simulink model "Assignment_2_Spatial_Robotics"  (R2024b)
settings: Solver=ode4  StartTime=0.0  StopTime=inf  FixedStep=0.01  RelTol=1e-3  EnableMultiTasking=on
libraries: sharedutil x10, vrlib x3, matrix_library x1
settings Model: Creator=Member  LastModifiedBy=adyak
settings SolverCC: AlgebraicLoopSolver=TrustRegion
settings DataIOCC: LimitDataPoints=on  SaveFormat=Array  SignalLoggingSaveFormat=ModelDataLogs  SaveOutput=off  SignalLogging=off  SaveTime=off  ReturnWorkspaceOutputs=off
settings OptimizationCC: ExpressionDepthLimit=2147483647  InitFltsAndDblsToZero=on  LifeSpan=inf
settings DebuggingCC: ReadBeforeWriteMsg=DisableAll  WriteAfterWriteMsg=DisableAll  WriteAfterReadMsg=DisableAll  SaveWithParameterizedLinksMsg=none  UnderspecifiedInitializationDetection=Classic  MergeDetectMultiDrivingBlocksExec=none  SolverPrmCheckMsg=warning  MultiTaskDSMMsg=none  MultiTaskCondExecSysMsg=none  FcnCallInpInsideContextMsg=warning  UnconnectedInputMsg=warning  UnconnectedOutputMsg=warning  UnconnectedLineMsg=warning  StateNameClashWarn=warning  SFUnexpectedBacktrackingDiag=warning  SFNoUnconditionalDefaultTransitionDiag=warning  SFExecutionAtInitializationDiag=none  ArithmeticOperatorsInVariantConditions=warning
settings HardwareCC: ProdBitPerPointer=32  ProdBitPerSizeT=32  ProdBitPerPtrDiffT=32  ProdLargestAtomicFloat=None  ProdIntDivRoundTo=Undefined  ProdEndianess=Unspecified  ProdWordSize=32  ProdHWDeviceType=32-bit Generic
settings ModelReferenceCC: UpdateModelReferenceTargets=IfOutOfDate  EnableRefExpFcnMdlSchedulingChecks=on  PropagateSignalLabelsOutOfModel=off
settings SFSimCC: SFSimEcho=off  CustomCodeUndefinedFunction=UseInterfaceOnly
settings RTWCC: GPUComputeCapability=3.5
settings CodeAppCC: StateflowObjectComments=on
settings GRTTargetCC: TargetFcnLib=ansi_tfl_tmw.mat  TargetLangStandard=C89/C90 (ANSI)  CombineOutputUpdateFcns=off  GRTInterface=on
settings ConfigComp: CovMetricSettings=dw  CovSaveCumulativeToWorkspaceVar=on  CovSaveSingleToWorkspaceVar=on

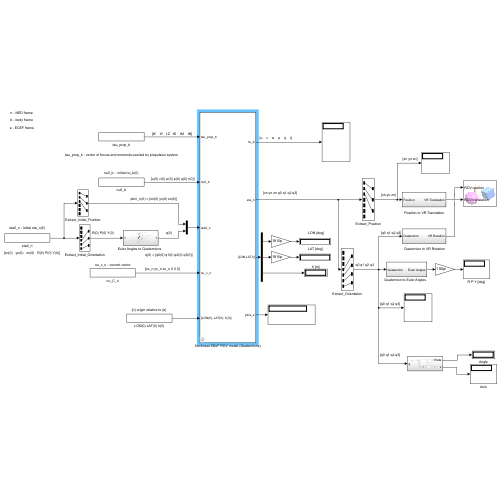
[thumbnail: Simulink's stored preview of the top-level diagram]
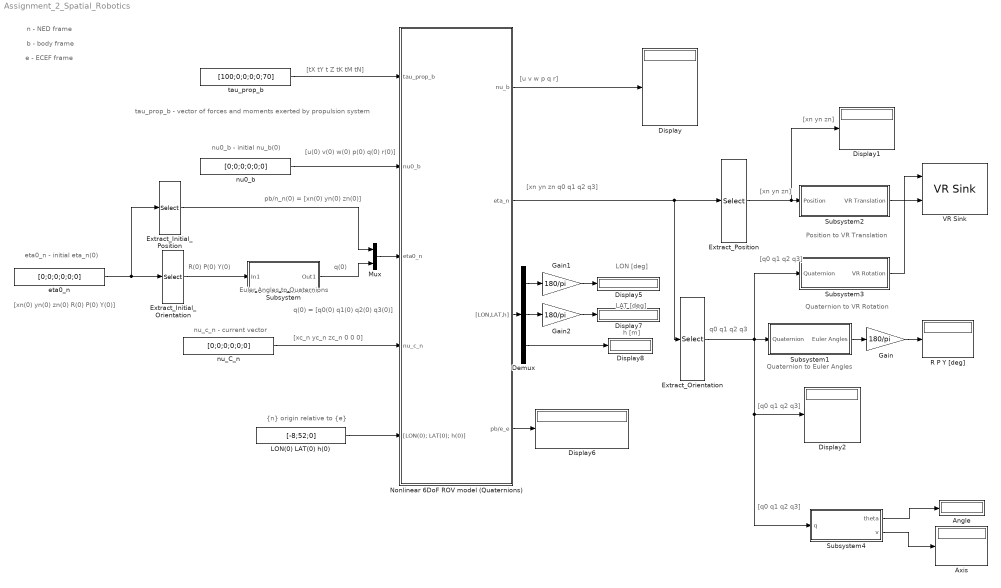
== system Assignment_2_Spatial_Robotics ==
  note: h [m]
  note: LON [deg]
  note: {n} origin relative to {e}
  note: q0 q1 q2 q3
  note: [xn yn zn]
  note: [xc_n yc_n zc_n 0 0 0]
  note: q(0)
  note: q(0) = [q0(0) q1(0) q2(0) q3(0)]
  note: pb/n_n(0) = [xn(0) yn(0) zn(0)]
  note: [u(0) v(0) w(0) p(0) q(0) r(0)]
  note: e - ECEF frame
  note: b - body frame
  note: n - NED frame
  note: tau_prop_b - vector of forces and moments exerted by propulsion system
  note: nu0_b - initial nu_b(0)
  note: eta0_n - initial eta_n(0)
  note: nu_c_n - current vector
  note: [tX tY t Z tK tM tN]
  note: [xn(0) yn(0) zn(0) R(0) P(0) Y(0)]
  note: [u v w p q r]
  note: [xn yn zn q0 q1 q2 q3]
  note: Euler Angles to Quaternions
  note: Quaternion to Euler Angles
  note: Quaternion to VR Rotation
  note: Position to VR Translation
  note: R(0) P(0) Y(0)
  note: [q0 q1 q2 q3]
  note: [xn yn zn]
  note: [q0 q1 q2 q3]
  note: [q0 q1 q2 q3]
  note: LAT [deg]
  Angle : Display
  Axis : Display
  Demux : Demux  Outputs=3
  Display{,1..2,5..8} (7 alike) : Display
  Extract_Initial_Orientation : Selector  InputPortWidth=6  IndexOptions=Index vector (dialog)  Indices=[4 5 6]  OutputSizes=1
  Extract_Initial_Position : Selector  InputPortWidth=6  IndexOptions=Index vector (dialog)  Indices=[1 2 3]  OutputSizes=1
  Extract_Orientation : Selector  InputPortWidth=7  IndexOptions=Index vector (dialog)  Indices=[4 5 6 7]  OutputSizes=1
  Extract_Position : Selector  InputPortWidth=7  IndexOptions=Index vector (dialog)  Indices=[1 2 3]  OutputSizes=1
  Gain : Gain  Gain=180/pi
  Gain1 : Gain  Gain=180/pi
  Gain2 : Gain  Gain=180/pi
  LON(0) LAT(0) h(0) : Constant  Value=[-8;52;0]
  Mux : Mux  Inputs=2
  Nonlinear 6DoF ROV model (Quaternions) : Subsystem  mask{Ig=[25 10 10;10 50 10;10 10 50], m=50, W=500, B=500, rG_b=[0;0;0], rB_b=[0;0;-0.1], MA=-diag([-30;-80;-80;-15;-30;-30]), DL=-diag([-200;-200;-200;-400;-300;-300]), dQ=-([-20;-20;-20;-10;-10;-10])}
      mask prompts: Ig "Inertia Tensor:"; m "Mass:"; W "Weigth:"; B "Buoyancy:"; MA "Added Mass Matrix MA:"; DL "Linear Damping Matrix DL:"; dQ "Quadratic Damping Vector dQ:"
      mask init:
      | Ib = Ig-m*skewsymm(rG_b)*skewsymm(rG_b);
      | MRB = [m*eye(3,3) -m*skewsymm(rG_b); m*skewsymm(rG_b) Ib];
      | M = MRB + MA;
      | inv_M = inv(M);
      | M11=MA(1:3,1:3);    M12=MA(1:3,4:6);
      | M21=MA(4:6,1:3);    M22=MA(4:6,4:6);
  R P Y [deg] : Display
  Subsystem : Subsystem
  Subsystem1 : Subsystem
  Subsystem2 : Subsystem
  Subsystem3 : Subsystem
  Subsystem4 : Subsystem
  VR Sink : vrlib/VR Sink  InstantiateOnLoad=on  SampleTime=-1  ViewEnable=on  RemoteChange=off  RemoteView=on  FieldsWritten=ROV.rotation.4.1.1.double#ROV.translation.3.1.1.double  WorldFileName=FALCON_test.wrl  AutoView=off  VideoDimensions=[]  AllowVariableSize=off  FigureProperties="{'Position', 'Name', 'Viewpoint', 'CameraBound', 'CameraDirection', 'CameraPosition', 'CameraUpVector', 'ZoomFactor', 'Antialiasing', 'Headlight', 'Lighting', 'Sound', 'StatusBar', 'Stereo3D', 'Stereo3DCameraOffset', 'Stereo3DHIT', 'ToolBar', 'Textures', 'Transparency', 'Triad', 'Wireframe', 'NavZones', 'NavMode', 'NavSpeed', 'CaptureFileFormat', 'CaptureFileName', 'Record2DCompressMethod', 'Record2DCompressQuality', 'Record2D', 'Record2DFileName', 'Record2DFPS', 'NavPanel'; [5.5850000000000000e+03   1.9000000000000000e+02   5.7600000000000000e+02   3.5000000000000000e+02], '', 'ONBOARD_CAMERA', 'on', [0.0000000000000000e+00   0.0000000000000000e+00  -1.0000000000000000e+00], [0.0000000000000000e+00   0.0000000000000000e+00   0.0000000000000000e+00], [0.0000000000000000e+00   1.0000000000000000e+00   0.0000000000000000e+00], [1.0000000000000000e+00], 'on', 'on', 'on', 'on', 'on', 'off', [1.0000000149011612e-01], [0.0000000000000000e+00], 'on', 'on', 'on', 'none', 'off', 'off', 'fly', 'normal', 'tif', '%f_anim_%n.tif', 'auto', [7.5000000000000000e+01], 'off', '%f_anim_%n.avi', 'auto', 'halfbar'}"
  eta0_n : Constant  Value=[0;0;0;0;0;0]
  nu0_b : Constant  Value=[0;0;0;0;0;0]
  nu_C_n : Constant  Value=[0;0;0;0;0;0]
  tau_prop_b : Constant  Value=[100;0;0;0;0;70]
  wires:
  nu0_b/1 -> Nonlinear 6DoF ROV model (Quaternions)/2(nu0_b)
  nu_C_n/1 -> Nonlinear 6DoF ROV model (Quaternions)/4(nu_c_n)
  tau_prop_b/1 -> Nonlinear 6DoF ROV model (Quaternions)/1(tau_prop_b)
  Nonlinear 6DoF ROV model (Quaternions)/2(eta_n) -> Extract_Orientation/1, Extract_Position/1
  Extract_Orientation/1 -> Subsystem4/1(q), Display2/1, Subsystem3/1(Quaternion), Subsystem1/1(Quaternion)
  Subsystem1/1(Euler Angles) -> Gain/1
  Gain/1 -> R P Y [deg]/1
  eta0_n/1 -> Extract_Initial_Position/1, Extract_Initial_Orientation/1
  Extract_Initial_Orientation/1 -> Subsystem/1(In1)
  Mux/1 -> Nonlinear 6DoF ROV model (Quaternions)/3(eta0_n)
  Subsystem/1(Out1) -> Mux/2
  Extract_Initial_Position/1 -> Mux/1
  Extract_Position/1 -> Display1/1, Subsystem2/1(Position)
  Subsystem3/1(VR Rotation) -> VR Sink/1
  Subsystem2/1(VR Translation) -> VR Sink/2
  Nonlinear 6DoF ROV model (Quaternions)/1(nu_b) -> Display/1
  Nonlinear 6DoF ROV model (Quaternions)/4(pb/e_e) -> Display6/1
  LON(0) LAT(0) h(0)/1 -> Nonlinear 6DoF ROV model (Quaternions)/5("[LON(0); LAT(0); h(0)]")
  Nonlinear 6DoF ROV model (Quaternions)/3("[LON,LAT,h]") -> Demux/1
  Demux/1 -> Gain1/1
  Gain1/1 -> Display5/1
  Gain2/1 -> Display7/1
  Demux/2 -> Gain2/1
  Demux/3 -> Display8/1
  Subsystem4/1(theta) -> Angle/1
  Subsystem4/2(v) -> Axis/1

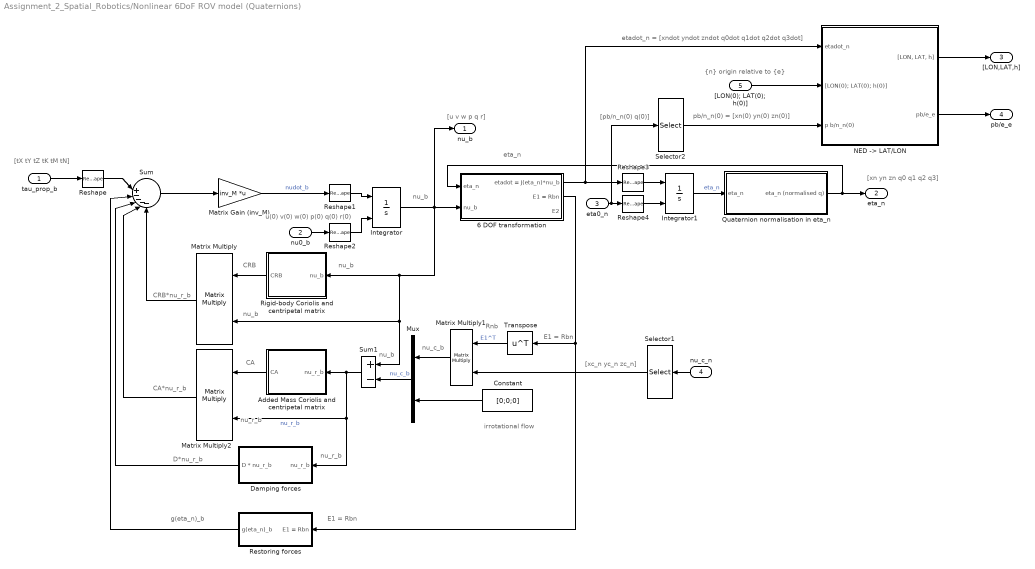
== system Assignment_2_Spatial_Robotics/Nonlinear 6DoF ROV model (Quaternions) ==
  note: irrotational flow
  note: etadot_n = [xndot yndot zndot q0dot q1dot q2dot q3dot]
  note: CA*nu_r_b
  note: D*nu_r_b
  note: g(eta_n)_b
  note: CRB
  note: CA
  note: u(0) v(0) w(0) p(0) q(0) r(0)
  note: eta_n
  note: [xn yn zn q0 q1 q2 q3]
  note: nu_r_b
  note: nu_c_b
  note: [xc_n yc_n zc_n]
  note: Rnb
  note: [tX tY tZ tK tM tN]
  note: [u v w p q r]
  note: nu_b
  note: E1 = Rbn
  note: nu_b
  note: nu_b
  note: nu_b
  note: nu_r_b
  note: CRB*nu_r_b
  note: pb/n_n(0) = [xn(0) yn(0) zn(0)]
  note: [pb/n_n(0) q(0)]
  note: {n} origin relative to {e}
  note: E1 = Rbn
  tau_prop_b : Inport
  nu0_b : Inport  Port=2
  eta0_n : Inport  Port=3
  nu_c_n : Inport  Port=4
  "[LON(0); LAT(0); h(0)]" : Inport  Port=5
  6 DOF transformation : Subsystem  AncestorBlock=MarineGNC/Library blocks/Axes transformations/6 DOF transformation
  Added Mass Coriolis and centripetal matrix : Subsystem
  Constant : Constant  Value=[0;0;0]
  Damping forces : Subsystem
  Integrator : Integrator  InitialConditionSource=external
  Integrator1 : Integrator  InitialConditionSource=external
  Matrix Gain (inv_M) : Gain  Gain=inv_M  Multiplication=Matrix(K*u)  SaturateOnIntegerOverflow=on  OutDataTypeStr=Inherit: Same as input  ParamDataTypeStr=Inherit: Same as input
  Matrix Multiply : Product  Multiplication=Matrix(*)
  Matrix Multiply1 : Product  Multiplication=Matrix(*)
  Matrix Multiply2 : Product  Multiplication=Matrix(*)
  Mux : Mux  Inputs=2
  "NED -> LAT/LON" : Subsystem
  Quaternion normalisation in eta_n : Subsystem
  Reshape{,1..4} (5 alike) : Reshape  OutputDimensionality=Column vector (2-D)
  Restoring forces : Subsystem
  Rigid-body Coriolis and centripetal matrix : Subsystem
  Selector1 : Selector  InputPortWidth=6  IndexOptions=Index vector (dialog)  Indices=[1 2 3]  OutputSizes=1
  Selector2 : Selector  InputPortWidth=7  IndexOptions=Index vector (dialog)  Indices=[1 2 3]  OutputSizes=1
  Sum : Sum  Inputs=|||+----  SaturateOnIntegerOverflow=on
  Sum1 : Sum  Inputs=+-
  Transpose : Math  Operator=transpose  SignedPower=on
  nu_b : Outport  VectorParamsAs1DForOutWhenUnconnected=off
  eta_n : Outport  Port=2  VectorParamsAs1DForOutWhenUnconnected=off
  "[LON,LAT,h]" : Outport  Port=3  VectorParamsAs1DForOutWhenUnconnected=off
  pb/e_e : Outport  Port=4  VectorParamsAs1DForOutWhenUnconnected=off
  wires:
  Matrix Multiply2/1 -> Sum/4
  Added Mass Coriolis and centripetal matrix/1(CA) -> Matrix Multiply2/1
  Sum1/1 -> Damping forces/1(nu_r_b), Matrix Multiply2/2, Added Mass Coriolis and centripetal matrix/1(nu_r_b)  "nu_r_b"
  Transpose/1 -> Matrix Multiply1/1  "E1^T"
  Matrix Multiply/1 -> Sum/5
  Rigid-body Coriolis and centripetal matrix/1(CRB) -> Matrix Multiply/1
  Reshape4/1 -> Integrator1/2
  Reshape3/1 -> Integrator1/1
  Reshape2/1 -> Integrator/2
  Reshape1/1 -> Integrator/1
  Reshape/1 -> Sum/1
  Restoring forces/1(g(eta_n)_b) -> Sum/2
  Damping forces/1(D * nu_r_b) -> Sum/3
  eta0_n/1 -> Selector2/1, Reshape4/1
  6 DOF transformation/1(etadot = J(eta_n)*nu_b) -> "NED -> LAT/LON"/1(etadot_n), Reshape3/1
  Integrator/1 -> 6 DOF transformation/2(nu_b), nu_b/1, Rigid-body Coriolis and centripetal matrix/1(nu_b), Matrix Multiply/2, Sum1/1
  nu0_b/1 -> Reshape2/1
  Matrix Gain (inv_M)/1 -> Reshape1/1  "nudot_b"
  Sum/1 -> Matrix Gain (inv_M)/1
  tau_prop_b/1 -> Reshape/1
  Matrix Multiply1/1 -> Mux/1
  Mux/1 -> Sum1/2  "nu_c_b"
  nu_c_n/1 -> Selector1/1
  Selector1/1 -> Matrix Multiply1/2
  6 DOF transformation/2(E1 = Rbn) -> Transpose/1, Restoring forces/1(E1 = Rbn)
  Integrator1/1 -> Quaternion normalisation in eta_n/1(eta_n)  "eta_n"
  Quaternion normalisation in eta_n/1(eta_n (normalised q)) -> 6 DOF transformation/1(eta_n), eta_n/1
  Constant/1 -> Mux/2
  Selector2/1 -> "NED -> LAT/LON"/3(p b/n_n(0))
  "[LON(0); LAT(0); h(0)]"/1 -> "NED -> LAT/LON"/2("[LON(0); LAT(0); h(0)]")
  "NED -> LAT/LON"/1("[LON, LAT, h]") -> "[LON,LAT,h]"/1
  "NED -> LAT/LON"/2(pb/e_e) -> pb/e_e/1

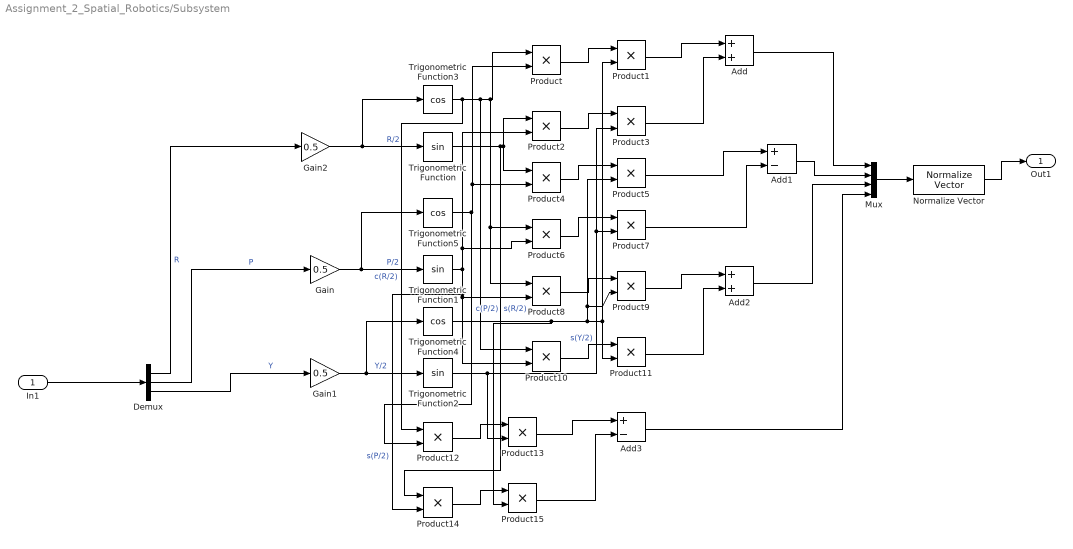
== system Assignment_2_Spatial_Robotics/Subsystem ==
  In1 : Inport
  Add : Sum
  Add1 : Sum  Inputs=+-
  Add2 : Sum
  Add3 : Sum  Inputs=+-
  Demux : Demux  Outputs=3
  Gain : Gain  Gain=0.5
  Gain1 : Gain  Gain=0.5
  Gain2 : Gain  Gain=0.5
  Mux : Mux
  Normalize Vector : vrlib/Utilities/Normalize Vector  maxzero=0
  Product{,1..15} (16 alike) : Product
  Trigonometric Function : Trigonometry
  Trigonometric Function1 : Trigonometry
  Trigonometric Function2 : Trigonometry
  Trigonometric Function3 : Trigonometry  Operator=cos
  Trigonometric Function4 : Trigonometry  Operator=cos
  Trigonometric Function5 : Trigonometry  Operator=cos
  Out1 : Outport
  wires:
  In1/1 -> Demux/1
  Demux/3 -> Gain1/1  "Y"
  Demux/2 -> Gain/1  "P"
  Demux/1 -> Gain2/1  "R"
  Gain1/1 -> Trigonometric Function4/1, Trigonometric Function2/1  "Y/2"
  Gain/1 -> Trigonometric Function5/1, Trigonometric Function1/1  "P/2"
  Gain2/1 -> Trigonometric Function3/1, Trigonometric Function/1  "R/2"
  Trigonometric Function/1 -> Product14/1, Product2/1, Product4/1  "s(R/2)"
  Trigonometric Function1/1 -> Product14/2, Product10/2, Product8/2, Product6/2, Product2/2  "s(P/2)"
  Product/1 -> Product1/1
  Trigonometric Function2/1 -> Product13/2, Product7/2, Product3/2  "s(Y/2)"
  Trigonometric Function3/1 -> Product12/1, Product10/1, Product8/1, Product6/1, Product/1  "c(R/2)"
  Trigonometric Function5/1 -> Product12/2, Product4/2, Product/2  "c(P/2)"
  Trigonometric Function4/1 -> Product15/2, Product9/2, Product5/2, Product11/2, Product1/2
  Product1/1 -> Add/1
  Product3/1 -> Add/2
  Product2/1 -> Product3/1
  Product5/1 -> Add1/1
  Product4/1 -> Product5/1
  Product7/1 -> Add1/2
  Product6/1 -> Product7/1
  Product9/1 -> Add2/1
  Product8/1 -> Product9/1
  Product11/1 -> Add2/2
  Product10/1 -> Product11/1
  Product13/1 -> Add3/1
  Product12/1 -> Product13/1
  Product15/1 -> Add3/2
  Product14/1 -> Product15/1
  Add/1 -> Mux/1
  Add1/1 -> Mux/2
  Add2/1 -> Mux/3
  Add3/1 -> Mux/4
  Mux/1 -> Normalize Vector/1
  Normalize Vector/1 -> Out1/1

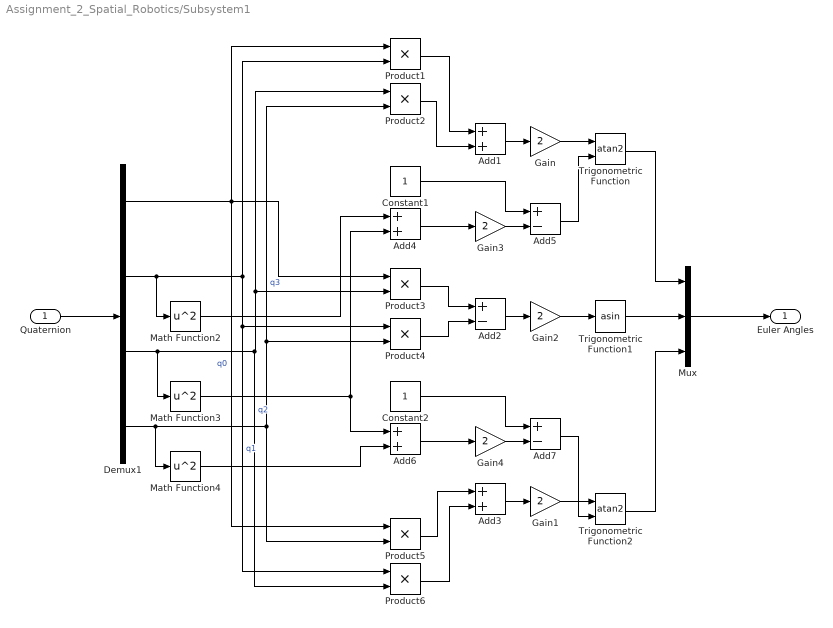
== system Assignment_2_Spatial_Robotics/Subsystem1 ==
  Quaternion : Inport
  Add{1,3..4,6} (4 alike) : Sum
  Add2 : Sum  Inputs=+-
  Add5 : Sum  Inputs=+-
  Add7 : Sum  Inputs=+-
  Constant1 : Constant
  Constant2 : Constant
  Demux1 : Demux
  Gain{,1..4} (5 alike) : Gain  Gain=2
  Math Function2 : Math  Operator=square  SignedPower=on
  Math Function3 : Math  Operator=square  SignedPower=on
  Math Function4 : Math  Operator=square  SignedPower=on
  Mux : Mux  Inputs=3
  Product{1..6} (6 alike) : Product
  Trigonometric Function : Trigonometry  Operator=atan2
  Trigonometric Function1 : Trigonometry  Operator=asin
  Trigonometric Function2 : Trigonometry  Operator=atan2
  Euler Angles : Outport  VectorParamsAs1DForOutWhenUnconnected=off
  wires:
  Quaternion/1 -> Demux1/1
  Demux1/1 -> Product5/1, Product3/1, Product1/1  "q0"
  Demux1/2 -> Product6/1, Product4/1, Product1/2, Math Function2/1  "q1"
  Demux1/3 -> Product6/2, Product3/2, Product2/1, Math Function3/1  "q2"
  Demux1/4 -> Product5/2, Product4/2, Product2/2, Math Function4/1  "q3"
  Trigonometric Function1/1 -> Mux/2
  Mux/1 -> Euler Angles/1
  Trigonometric Function/1 -> Mux/1
  Trigonometric Function2/1 -> Mux/3
  Gain/1 -> Trigonometric Function/1
  Gain1/1 -> Trigonometric Function2/1
  Gain2/1 -> Trigonometric Function1/1
  Add1/1 -> Gain/1
  Add2/1 -> Gain2/1
  Add3/1 -> Gain1/1
  Product3/1 -> Add2/1
  Product4/1 -> Add2/2
  Product5/1 -> Add3/1
  Product6/1 -> Add3/2
  Product2/1 -> Add1/2
  Product1/1 -> Add1/1
  Add4/1 -> Gain3/1
  Gain3/1 -> Add5/2
  Constant1/1 -> Add5/1
  Add5/1 -> Trigonometric Function/2
  Add7/1 -> Trigonometric Function2/2
  Add6/1 -> Gain4/1
  Gain4/1 -> Add7/2
  Constant2/1 -> Add7/1
  Math Function2/1 -> Add4/1
  Math Function3/1 -> Add6/1, Add4/2
  Math Function4/1 -> Add6/2

== system Assignment_2_Spatial_Robotics/Subsystem2 ==
  Position : Inport
  Demux : Demux  Outputs=3
  Gain : Gain  Gain=-1
  Gain1 : Gain  Gain=-1
  Mux : Mux  Inputs=3
  VR Translation : Outport  VectorParamsAs1DForOutWhenUnconnected=off
  wires:
  Position/1 -> Demux/1
  Demux/1 -> Gain/1  "x"
  Demux/2 -> Mux/1  "y"
  Demux/3 -> Gain1/1  "z"
  Mux/1 -> VR Translation/1
  Gain1/1 -> Mux/2
  Gain/1 -> Mux/3

== system Assignment_2_Spatial_Robotics/Subsystem3 ==
  Quaternion : Inport
  Demux1 : Demux
  Gain : Gain  Gain=2
  Gain1 : Gain  Gain=-1
  Gain2 : Gain  Gain=-1
  Mux : Mux
  Trigonometric Function : Trigonometry  Operator=acos
  VR Rotation : Outport  VectorParamsAs1DForOutWhenUnconnected=off
  wires:
  Trigonometric Function/1 -> Gain/1
  Gain/1 -> Mux/4
  Mux/1 -> VR Rotation/1
  Demux1/1 -> Trigonometric Function/1  "q0"
  Demux1/2 -> Gain1/1  "q1"
  Demux1/3 -> Mux/1  "q2"
  Demux1/4 -> Gain2/1  "q3"
  Gain2/1 -> Mux/2
  Gain1/1 -> Mux/3
  Quaternion/1 -> Demux1/1

== system Assignment_2_Spatial_Robotics/Subsystem4 ==
  q : Inport
  Demux : Demux
  Gain : Gain  Gain=2
  Mux : Mux  Inputs=3
  Normalize Vector : vrlib/Utilities/Normalize Vector  maxzero=0
  Product : Product
  Trigonometric Function : Trigonometry  Operator=cos
  theta : Outport
  v : Outport  Port=2
  wires:
  q/1 -> Demux/1
  Demux/1 -> Trigonometric Function/1  "q0"
  Trigonometric Function/1 -> Product/1
  Gain/1 -> Product/2
  Demux/2 -> Mux/1  "q1"
  Demux/3 -> Mux/2  "q2"
  Demux/4 -> Mux/3  "q3"
  Mux/1 -> Normalize Vector/1
  Normalize Vector/1 -> v/1
  Product/1 -> theta/1

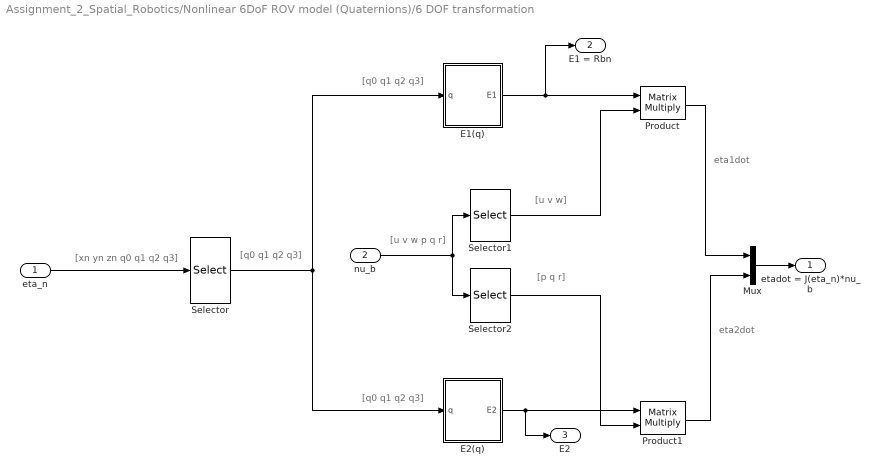
== system Assignment_2_Spatial_Robotics/Nonlinear 6DoF ROV model (Quaternions)/6 DOF transformation ==
  note: [u v w p q r]
  note: [q0 q1 q2 q3]
  note: [xn yn zn q0 q1 q2 q3]
  note: eta1dot
  note: eta2dot
  note: [q0 q1 q2 q3]
  note: [q0 q1 q2 q3]
  note: [u v w]
  note: [p q r]
  eta_n : Inport
  nu_b : Inport  Port=2
  E1(q) : Subsystem
  E2(q) : Subsystem
  Mux : Mux  Inputs=2
  Product : Product  Inputs=**  Multiplication=Matrix(*)  SaturateOnIntegerOverflow=on  OutDataTypeStr=Inherit: Same as first input
  Product1 : Product  Inputs=**  Multiplication=Matrix(*)  SaturateOnIntegerOverflow=on  OutDataTypeStr=Inherit: Same as first input
  Selector : Selector  InputPortWidth=7  IndexOptions=Index vector (dialog)  Indices=[4 5 6 7]  OutputSizes=1
  Selector1 : Selector  InputPortWidth=6  IndexOptions=Index vector (dialog)  Indices=[1 2 3]  OutputSizes=1
  Selector2 : Selector  InputPortWidth=6  IndexOptions=Index vector (dialog)  Indices=[4 5 6]  OutputSizes=1
  etadot = J(eta_n)*nu_b : Outport  VectorParamsAs1DForOutWhenUnconnected=off
  E1 = Rbn : Outport  Port=2  VectorParamsAs1DForOutWhenUnconnected=off
  E2 : Outport  Port=3  VectorParamsAs1DForOutWhenUnconnected=off
  wires:
  Product1/1 -> Mux/2
  Mux/1 -> etadot = J(eta_n)*nu_b/1
  Product/1 -> Mux/1
  E2(q)/1(E2) -> Product1/1, E2/1
  Selector2/1 -> Product1/2
  Selector1/1 -> Product/2
  nu_b/1 -> Selector2/1, Selector1/1
  E1(q)/1(E1) -> Product/1, E1 = Rbn/1
  eta_n/1 -> Selector/1
  Selector/1 -> E2(q)/1(q), E1(q)/1(q)

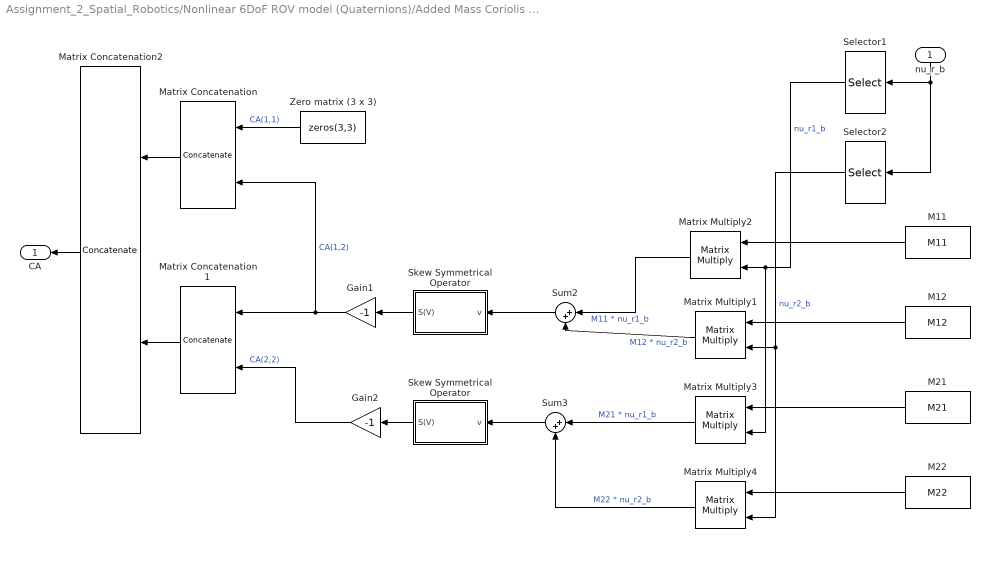
== system Assignment_2_Spatial_Robotics/Nonlinear 6DoF ROV model (Quaternions)/Added Mass Coriolis and centripetal matrix ==
  nu_r_b : Inport
  Gain1 : Gain  Gain=-1  SaturateOnIntegerOverflow=on  OutDataTypeStr=Inherit: Same as input  ParamDataTypeStr=Inherit: Same as input
  Gain2 : Gain  Gain=-1  SaturateOnIntegerOverflow=on  OutDataTypeStr=Inherit: Same as input  ParamDataTypeStr=Inherit: Same as input
  M11 : Constant  Value=M11
  M12 : Constant  Value=M12
  M21 : Constant  Value=M21
  M22 : Constant  Value=M22
  Matrix Concatenation : Concatenate  Mode=Multidimensional array
  Matrix Concatenation1 : Concatenate  Mode=Multidimensional array
  Matrix Concatenation2 : Concatenate  Mode=Multidimensional array  ConcatenateDimension=2
  Matrix Multiply{1..4} (4 alike) : Product  Multiplication=Matrix(*)
  Selector1 : Selector  InputPortWidth=6  IndexOptions=Index vector (dialog)  Indices=[1 2 3]  OutputSizes=1
  Selector2 : Selector  InputPortWidth=6  IndexOptions=Index vector (dialog)  Indices=[4 5 6]  OutputSizes=1
  Skew Symmetrical Operator : Subsystem
  "Skew Symmetrical Operator " : Subsystem
  Sum2 : Sum  Inputs=|++  SaturateOnIntegerOverflow=on
  Sum3 : Sum  Inputs=|++  SaturateOnIntegerOverflow=on
  Zero matrix (3 x 3) : Constant  Value=zeros(3,3)
  CA : Outport  VectorParamsAs1DForOutWhenUnconnected=off
  wires:
  Zero matrix (3 x 3)/1 -> Matrix Concatenation/1  "CA(1,1)"
  Matrix Concatenation/1 -> Matrix Concatenation2/1
  Matrix Concatenation1/1 -> Matrix Concatenation2/2
  Matrix Multiply2/1 -> Sum2/1  "M11 * nu_r1_b"
  Matrix Multiply1/1 -> Sum2/2  "M12 * nu_r2_b"
  Matrix Multiply3/1 -> Sum3/1  "M21 * nu_r1_b"
  Selector1/1 -> Matrix Multiply2/2, Matrix Multiply3/2  "nu_r1_b"
  Matrix Multiply4/1 -> Sum3/2  "M22 * nu_r2_b"
  Selector2/1 -> Matrix Multiply1/2, Matrix Multiply4/2  "nu_r2_b"
  Sum2/1 -> "Skew Symmetrical Operator "/1(v)
  Sum3/1 -> Skew Symmetrical Operator/1(v)
  "Skew Symmetrical Operator "/1(S(V)) -> Gain1/1
  Skew Symmetrical Operator/1(S(V)) -> Gain2/1
  Gain1/1 -> Matrix Concatenation1/1, Matrix Concatenation/2  "CA(1,2)"
  Gain2/1 -> Matrix Concatenation1/2  "CA(2,2)"
  nu_r_b/1 -> Selector1/1, Selector2/1
  Matrix Concatenation2/1 -> CA/1
  M11/1 -> Matrix Multiply2/1
  M12/1 -> Matrix Multiply1/1
  M21/1 -> Matrix Multiply3/1
  M22/1 -> Matrix Multiply4/1

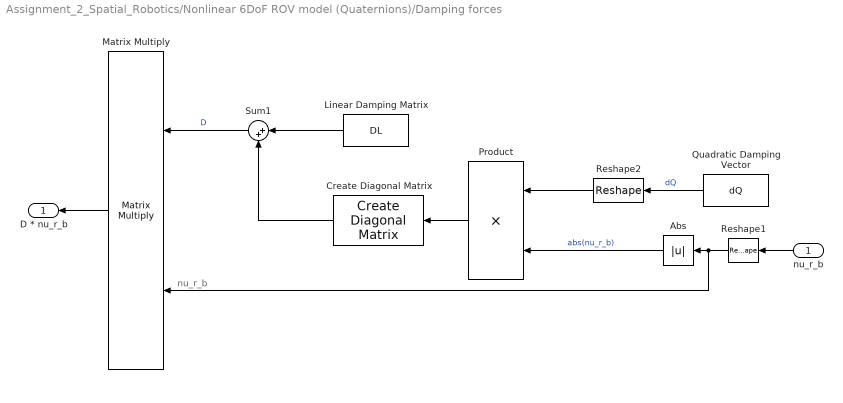
== system Assignment_2_Spatial_Robotics/Nonlinear 6DoF ROV model (Quaternions)/Damping forces ==
  note: nu_r_b
  nu_r_b : Inport
  Abs : Abs
  Create Diagonal Matrix : matrix_library/Create Diagonal Matrix
  Linear Damping Matrix : Constant  Value=DL
  Matrix Multiply : Product  Multiplication=Matrix(*)
  Product : Product  SaturateOnIntegerOverflow=on  OutDataTypeStr=Inherit: Same as first input
  Quadratic Damping Vector : Constant  Value=dQ
  Reshape1 : Reshape  OutputDimensionality=Column vector (2-D)
  Reshape2 : Reshape  OutputDimensionality=Column vector (2-D)  OutputDimensions=[6,6]
  Sum1 : Sum  Inputs=|++  SaturateOnIntegerOverflow=on
  D * nu_r_b : Outport  VectorParamsAs1DForOutWhenUnconnected=off
  wires:
  Reshape2/1 -> Product/1
  Reshape1/1 -> Matrix Multiply/2, Abs/1
  Matrix Multiply/1 -> D * nu_r_b/1
  Sum1/1 -> Matrix Multiply/1  "D"
  nu_r_b/1 -> Reshape1/1
  Linear Damping Matrix/1 -> Sum1/1
  Create Diagonal Matrix/1 -> Sum1/2
  Product/1 -> Create Diagonal Matrix/1
  Abs/1 -> Product/2  "abs(nu_r_b)"
  Quadratic Damping Vector/1 -> Reshape2/1  "dQ"

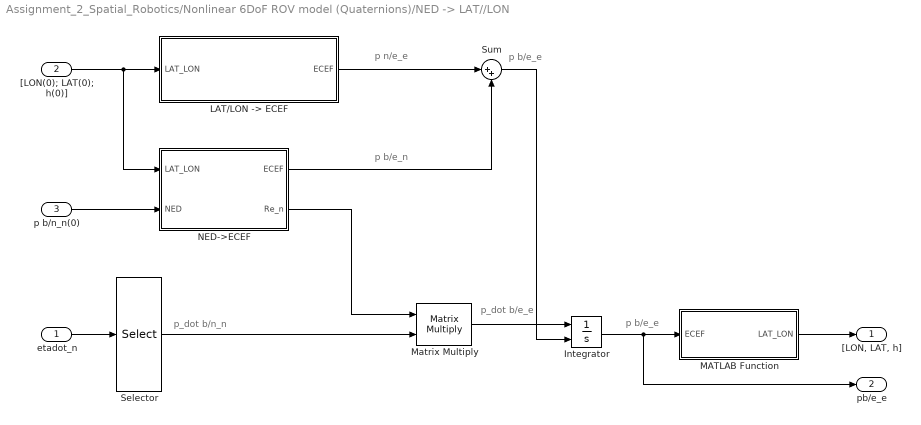
== system Assignment_2_Spatial_Robotics/Nonlinear 6DoF ROV model (Quaternions)/NED -> LAT//LON ==
  note: p_dot b/n_n
  note: p_dot b/e_e
  note: p b/e_e
  note: p n/e_e
  note: p b/e_n
  note: p b/e_e
  etadot_n : Inport
  "[LON(0); LAT(0); h(0)]" : Inport  Port=2
  p b/n_n(0) : Inport  Port=3
  Integrator : Integrator  InitialConditionSource=external
  "LAT/LON -> ECEF" : MATLAB Function  TreatAsAtomicUnit=on
  MATLAB Function : MATLAB Function  TreatAsAtomicUnit=on
  Matrix Multiply : Product  Multiplication=Matrix(*)
  NED->ECEF : MATLAB Function  TreatAsAtomicUnit=on
  Selector : Selector  InputPortWidth=7  IndexOptions=Index vector (dialog)  Indices=[1 2 3]  OutputSizes=1
  Sum : Sum  Inputs=|++
  "[LON, LAT, h]" : Outport
  pb/e_e : Outport  Port=2
  wires:
  etadot_n/1 -> Selector/1
  Selector/1 -> Matrix Multiply/2
  "[LON(0); LAT(0); h(0)]"/1 -> NED->ECEF/1(LAT_LON), "LAT/LON -> ECEF"/1(LAT_LON)
  Sum/1 -> Integrator/2
  Integrator/1 -> MATLAB Function/1(ECEF), pb/e_e/1
  MATLAB Function/1(LAT_LON) -> "[LON, LAT, h]"/1
  p b/n_n(0)/1 -> NED->ECEF/2(NED)
  Matrix Multiply/1 -> Integrator/1
  NED->ECEF/2(Re_n) -> Matrix Multiply/1
  NED->ECEF/1(ECEF) -> Sum/2
  "LAT/LON -> ECEF"/1(ECEF) -> Sum/1

== system Assignment_2_Spatial_Robotics/Nonlinear 6DoF ROV model (Quaternions)/Quaternion normalisation in eta_n ==
  note: q (normalised)
  note: q
  note: norm(q)
  note: q=[q0 q1 q2 q3]
  note: [xn yn zn]
  note: [xn yn zn q0 q1 q2 q3]
  eta_n : Inport
  Mux : Mux  Inputs=2
  Product : Product  Inputs=*/  SaturateOnIntegerOverflow=on  OutDataTypeStr=Inherit: Same as first input
  Reshape : Reshape  OutputDimensionality=Column vector (2-D)
  Selector : Selector  InputPortWidth=7  IndexOptions=Index vector (dialog)  Indices=[1 2 3]  OutputSizes=1
  Selector1 : Selector  InputPortWidth=7  IndexOptions=Index vector (dialog)  Indices=[4 5 6 7]  OutputSizes=1
  norm : MATLABFcn  MATLABFcn=norm  OutputDimensions=1
  eta_n (normalised q) : Outport  VectorParamsAs1DForOutWhenUnconnected=off
  wires:
  eta_n/1 -> Selector1/1, Selector/1
  Selector1/1 -> norm/1, Product/1
  norm/1 -> Product/2
  Selector/1 -> Mux/1
  Product/1 -> Mux/2
  Mux/1 -> Reshape/1
  Reshape/1 -> eta_n (normalised q)/1

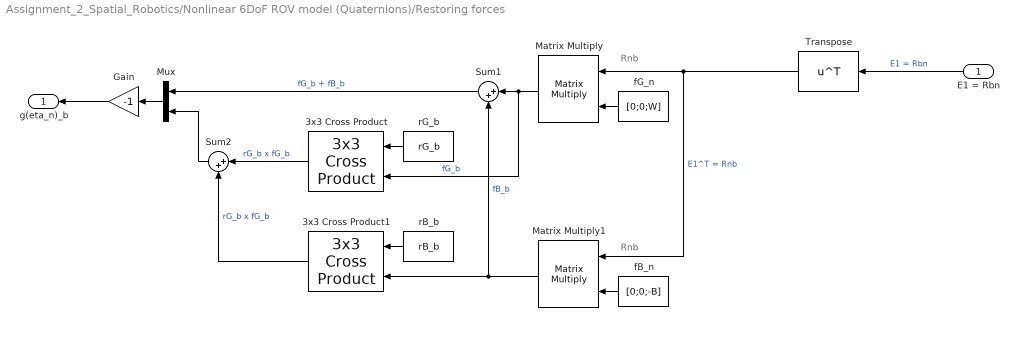
== system Assignment_2_Spatial_Robotics/Nonlinear 6DoF ROV model (Quaternions)/Restoring forces ==
  note: Rnb
  note: Rnb
  E1 = Rbn : Inport
  3x3 Cross Product : sharedutil/3x3 Cross Product  aMode=aMode
  3x3 Cross Product1 : sharedutil/3x3 Cross Product  aMode=aMode
  Gain : Gain  Gain=-1  SaturateOnIntegerOverflow=on  OutDataTypeStr=Inherit: Same as input  ParamDataTypeStr=Inherit: Same as input
  Matrix Multiply : Product  Multiplication=Matrix(*)
  Matrix Multiply1 : Product  Multiplication=Matrix(*)
  Mux : Mux  Inputs=2
  Sum1 : Sum  Inputs=|++  SaturateOnIntegerOverflow=on
  Sum2 : Sum  Inputs=|++  SaturateOnIntegerOverflow=on
  Transpose : Math  Operator=transpose  SignedPower=on
  fB_n : Constant  Value=[0;0;-B]
  fG_n : Constant  Value=[0;0;W]
  rB_b : Constant  Value=rB_b
  rG_b : Constant  Value=rG_b
  g(eta_n)_b : Outport  VectorParamsAs1DForOutWhenUnconnected=off
  wires:
  E1 = Rbn/1 -> Transpose/1  "E1 = Rbn"
  Transpose/1 -> Matrix Multiply/1, Matrix Multiply1/1  "E1^T = Rnb"
  fG_n/1 -> Matrix Multiply/2
  fB_n/1 -> Matrix Multiply1/2
  Matrix Multiply/1 -> Sum1/1, 3x3 Cross Product/2  "fG_b"
  Matrix Multiply1/1 -> Sum1/2, 3x3 Cross Product1/2  "fB_b"
  rG_b/1 -> 3x3 Cross Product/1
  Sum1/1 -> Mux/1  "fG_b + fB_b"
  3x3 Cross Product/1 -> Sum2/1  "rG_b x fG_b"
  3x3 Cross Product1/1 -> Sum2/2  "rG_b x fG_b"
  rB_b/1 -> 3x3 Cross Product1/1
  Sum2/1 -> Mux/2
  Mux/1 -> Gain/1
  Gain/1 -> g(eta_n)_b/1

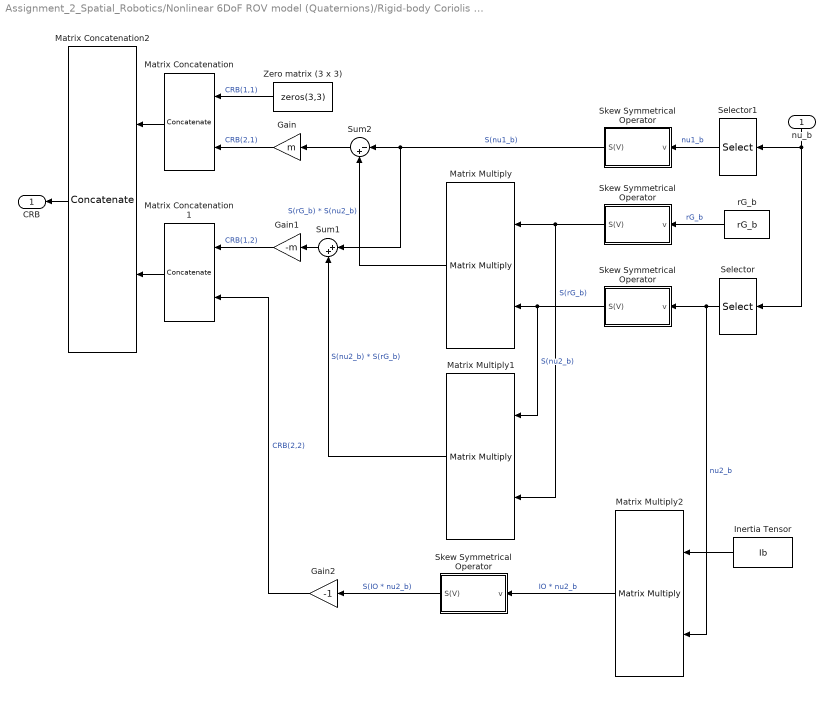
== system Assignment_2_Spatial_Robotics/Nonlinear 6DoF ROV model (Quaternions)/Rigid-body Coriolis and centripetal matrix ==
  nu_b : Inport
  Gain : Gain  Gain=m  SaturateOnIntegerOverflow=on  OutDataTypeStr=Inherit: Same as input  ParamDataTypeStr=Inherit: Same as input
  Gain1 : Gain  Gain=-m  SaturateOnIntegerOverflow=on  OutDataTypeStr=Inherit: Same as input  ParamDataTypeStr=Inherit: Same as input
  Gain2 : Gain  Gain=-1  SaturateOnIntegerOverflow=on  OutDataTypeStr=Inherit: Same as input  ParamDataTypeStr=Inherit: Same as input
  Inertia Tensor : Constant  Value=Ib
  Matrix Concatenation : Concatenate  Mode=Multidimensional array
  Matrix Concatenation1 : Concatenate  Mode=Multidimensional array
  Matrix Concatenation2 : Concatenate  Mode=Multidimensional array  ConcatenateDimension=2
  Matrix Multiply : Product  Multiplication=Matrix(*)
  Matrix Multiply1 : Product  Multiplication=Matrix(*)
  Matrix Multiply2 : Product  Multiplication=Matrix(*)
  Selector : Selector  InputPortWidth=6  IndexOptions=Index vector (dialog)  Indices=[4 5 6]  OutputSizes=1
  Selector1 : Selector  InputPortWidth=6  IndexOptions=Index vector (dialog)  Indices=[1 2 3]  OutputSizes=1
  "Skew Symmetrical Operator " : Subsystem
  Skew Symmetrical Operator : Subsystem
  "Skew Symmetrical Operator " : Subsystem
  "Skew Symmetrical Operator  " : Subsystem
  Sum1 : Sum  Inputs=|++  SaturateOnIntegerOverflow=on
  Sum2 : Sum  Inputs=|-+  SaturateOnIntegerOverflow=on
  Zero matrix (3 x 3) : Constant  Value=zeros(3,3)
  rG_b : Constant  Value=rG_b
  CRB : Outport  VectorParamsAs1DForOutWhenUnconnected=off
  wires:
  nu_b/1 -> Selector/1, Selector1/1
  Selector1/1 -> Skew Symmetrical Operator/1(v)  "nu1_b"
  Selector/1 -> "Skew Symmetrical Operator "/1(v), Matrix Multiply2/2  "nu2_b"
  rG_b/1 -> "Skew Symmetrical Operator  "/1(v)  "rG_b"
  Skew Symmetrical Operator/1(S(V)) -> Sum2/1, Sum1/1  "S(nu1_b)"
  "Skew Symmetrical Operator "/1(S(V)) -> Matrix Multiply/2, Matrix Multiply1/1  "S(nu2_b)"
  "Skew Symmetrical Operator  "/1(S(V)) -> Matrix Multiply/1, Matrix Multiply1/2  "S(rG_b)"
  Matrix Multiply/1 -> Sum2/2  "S(rG_b) * S(nu2_b)"
  Sum2/1 -> Gain/1
  Gain/1 -> Matrix Concatenation/2  "CRB(2,1)"
  Zero matrix (3 x 3)/1 -> Matrix Concatenation/1  "CRB(1,1)"
  Matrix Multiply1/1 -> Sum1/2  "S(nu2_b) * S(rG_b)"
  Sum1/1 -> Gain1/1
  Gain1/1 -> Matrix Concatenation1/1  "CRB(1,2)"
  Inertia Tensor/1 -> Matrix Multiply2/1
  Matrix Multiply2/1 -> "Skew Symmetrical Operator "/1(v)  "IO * nu2_b"
  "Skew Symmetrical Operator "/1(S(V)) -> Gain2/1  "S(IO * nu2_b)"
  Gain2/1 -> Matrix Concatenation1/2  "CRB(2,2)"
  Matrix Concatenation/1 -> Matrix Concatenation2/1
  Matrix Concatenation1/1 -> Matrix Concatenation2/2
  Matrix Concatenation2/1 -> CRB/1

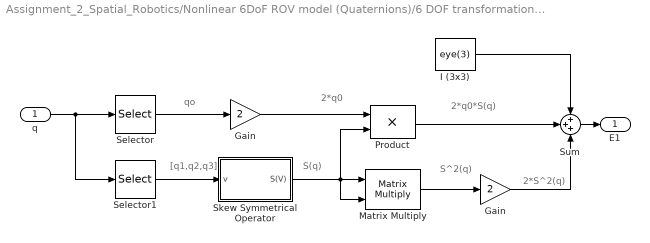
== system Assignment_2_Spatial_Robotics/Nonlinear 6DoF ROV model (Quaternions)/6 DOF transformation/E1(q) ==
  note: S(q)
  note: 2*q0
  note: [q1,q2,q3]
  note: qo
  note: S^2(q)
  note: 2*S^2(q)
  note: 2*q0*S(q)
  q : Inport
  Gain : Gain  Gain=2  SaturateOnIntegerOverflow=on  OutDataTypeStr=Inherit: Same as input  ParamDataTypeStr=Inherit: Same as input
  "Gain " : Gain  Gain=2  SaturateOnIntegerOverflow=on  OutDataTypeStr=Inherit: Same as input  ParamDataTypeStr=Inherit: Same as input
  I (3x3) : Constant  Value=eye(3)
  Matrix Multiply : Product  Multiplication=Matrix(*)
  Product : Product  SaturateOnIntegerOverflow=on  OutDataTypeStr=Inherit: Same as first input
  Selector : Selector  InputPortWidth=4  IndexOptions=Index vector (dialog)  Indices=[1]  OutputSizes=1
  Selector1 : Selector  InputPortWidth=4  IndexOptions=Index vector (dialog)  Indices=[2 3 4]  OutputSizes=1
  Skew Symmetrical Operator : Subsystem
  Sum : Sum  Inputs=+++  SaturateOnIntegerOverflow=on
  E1 : Outport  VectorParamsAs1DForOutWhenUnconnected=off
  wires:
  q/1 -> Selector/1, Selector1/1
  Selector/1 -> "Gain "/1
  Selector1/1 -> Skew Symmetrical Operator/1(v)
  Skew Symmetrical Operator/1(S(V)) -> Matrix Multiply/1, Matrix Multiply/2, Product/2
  Matrix Multiply/1 -> Gain/1
  "Gain "/1 -> Product/1
  I (3x3)/1 -> Sum/1
  Product/1 -> Sum/2
  Gain/1 -> Sum/3
  Sum/1 -> E1/1

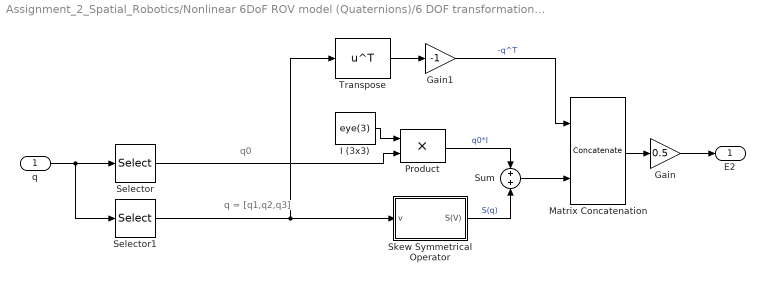
== system Assignment_2_Spatial_Robotics/Nonlinear 6DoF ROV model (Quaternions)/6 DOF transformation/E2(q) ==
  note: q = [q1,q2,q3]
  note: q0
  q : Inport
  Gain : Gain  Gain=0.5  SaturateOnIntegerOverflow=on  OutDataTypeStr=Inherit: Same as input  ParamDataTypeStr=Inherit: Same as input
  Gain1 : Gain  Gain=-1  SaturateOnIntegerOverflow=on  OutDataTypeStr=Inherit: Same as input  ParamDataTypeStr=Inherit: Same as input
  I (3x3) : Constant  Value=eye(3)
  Matrix Concatenation : Concatenate  Mode=Multidimensional array
  Product : Product  SaturateOnIntegerOverflow=on  OutDataTypeStr=Inherit: Same as first input
  Selector : Selector  InputPortWidth=4  IndexOptions=Index vector (dialog)  Indices=[1]  OutputSizes=1
  Selector1 : Selector  InputPortWidth=4  IndexOptions=Index vector (dialog)  Indices=[2 3 4]  OutputSizes=1
  Skew Symmetrical Operator : Subsystem
  Sum : Sum  SaturateOnIntegerOverflow=on
  Transpose : Math  Operator=transpose  SignedPower=on
  E2 : Outport  VectorParamsAs1DForOutWhenUnconnected=off
  wires:
  Selector1/1 -> Skew Symmetrical Operator/1(v), Transpose/1
  Selector/1 -> Product/2
  q/1 -> Selector1/1, Selector/1
  I (3x3)/1 -> Product/1
  Product/1 -> Sum/1  "q0*I"
  Skew Symmetrical Operator/1(S(V)) -> Sum/2  "S(q)"
  Transpose/1 -> Gain1/1
  Gain1/1 -> Matrix Concatenation/1  "-q^T"
  Sum/1 -> Matrix Concatenation/2
  Matrix Concatenation/1 -> Gain/1
  Gain/1 -> E2/1

== system Assignment_2_Spatial_Robotics/Nonlinear 6DoF ROV model (Quaternions)/Added Mass Coriolis and centripetal matrix/Skew Symmetrical Operator ==
  v : Inport
  Constant : Constant  Value=0
  Create 3x3 Matrix : sharedutil/Create 3x3 Matrix  aMode=aMode
  Demux : Demux  Outputs=3
      settings: DisplayOption=none
  Gain : Gain  Gain=-1  SaturateOnIntegerOverflow=on  OutDataTypeStr=Inherit: Same as input  ParamDataTypeStr=Inherit: Same as input
  Gain1 : Gain  Gain=-1  SaturateOnIntegerOverflow=on  OutDataTypeStr=Inherit: Same as input  ParamDataTypeStr=Inherit: Same as input
  Gain2 : Gain  Gain=-1  SaturateOnIntegerOverflow=on  OutDataTypeStr=Inherit: Same as input  ParamDataTypeStr=Inherit: Same as input
  S(V) : Outport  VectorParamsAs1DForOutWhenUnconnected=off
  wires:
  v/1 -> Demux/1
  Create 3x3 Matrix/1 -> S(V)/1
  Gain2/1 -> Create 3x3 Matrix/2  "-v(3)"
  Gain1/1 -> Create 3x3 Matrix/7  "-v(2)"
  Gain/1 -> Create 3x3 Matrix/6  "-v(1)"
  Demux/3 -> Create 3x3 Matrix/4, Gain2/1  "v(3)"
  Demux/2 -> Create 3x3 Matrix/3, Gain1/1  "v(2)"
  Demux/1 -> Create 3x3 Matrix/8, Gain/1  "v(1)"
  Constant/1 -> Create 3x3 Matrix/5, Create 3x3 Matrix/9, Create 3x3 Matrix/1

== system Assignment_2_Spatial_Robotics/Nonlinear 6DoF ROV model (Quaternions)/Added Mass Coriolis and centripetal matrix/Skew Symmetrical Operator  ==
  v : Inport
  Constant : Constant  Value=0
  Create 3x3 Matrix : sharedutil/Create 3x3 Matrix  aMode=aMode
  Demux : Demux  Outputs=3
      settings: DisplayOption=none
  Gain : Gain  Gain=-1  SaturateOnIntegerOverflow=on  OutDataTypeStr=Inherit: Same as input  ParamDataTypeStr=Inherit: Same as input
  Gain1 : Gain  Gain=-1  SaturateOnIntegerOverflow=on  OutDataTypeStr=Inherit: Same as input  ParamDataTypeStr=Inherit: Same as input
  Gain2 : Gain  Gain=-1  SaturateOnIntegerOverflow=on  OutDataTypeStr=Inherit: Same as input  ParamDataTypeStr=Inherit: Same as input
  S(V) : Outport  VectorParamsAs1DForOutWhenUnconnected=off
  wires:
  Constant/1 -> Create 3x3 Matrix/1, Create 3x3 Matrix/9, Create 3x3 Matrix/5
  Demux/1 -> Gain/1, Create 3x3 Matrix/8  "v(1)"
  Demux/2 -> Gain1/1, Create 3x3 Matrix/3  "v(2)"
  Demux/3 -> Gain2/1, Create 3x3 Matrix/4  "v(3)"
  Gain/1 -> Create 3x3 Matrix/6  "-v(1)"
  Gain1/1 -> Create 3x3 Matrix/7  "-v(2)"
  Gain2/1 -> Create 3x3 Matrix/2  "-v(3)"
  Create 3x3 Matrix/1 -> S(V)/1
  v/1 -> Demux/1

== system Assignment_2_Spatial_Robotics/Nonlinear 6DoF ROV model (Quaternions)/Rigid-body Coriolis and centripetal matrix/Skew Symmetrical Operator  ==
  v : Inport
  Constant : Constant  Value=0
  Create 3x3 Matrix : sharedutil/Create 3x3 Matrix  aMode=aMode
  Demux : Demux  Outputs=3
      settings: DisplayOption=none
  Gain : Gain  Gain=-1  SaturateOnIntegerOverflow=on  OutDataTypeStr=Inherit: Same as input  ParamDataTypeStr=Inherit: Same as input
  Gain1 : Gain  Gain=-1  SaturateOnIntegerOverflow=on  OutDataTypeStr=Inherit: Same as input  ParamDataTypeStr=Inherit: Same as input
  Gain2 : Gain  Gain=-1  SaturateOnIntegerOverflow=on  OutDataTypeStr=Inherit: Same as input  ParamDataTypeStr=Inherit: Same as input
  S(V) : Outport  VectorParamsAs1DForOutWhenUnconnected=off
  wires:
  Constant/1 -> Create 3x3 Matrix/1, Create 3x3 Matrix/9, Create 3x3 Matrix/5
  Demux/1 -> Gain/1, Create 3x3 Matrix/8  "v(1)"
  Demux/2 -> Gain1/1, Create 3x3 Matrix/3  "v(2)"
  Demux/3 -> Gain2/1, Create 3x3 Matrix/4  "v(3)"
  Gain/1 -> Create 3x3 Matrix/6  "-v(1)"
  Gain1/1 -> Create 3x3 Matrix/7  "-v(2)"
  Gain2/1 -> Create 3x3 Matrix/2  "-v(3)"
  Create 3x3 Matrix/1 -> S(V)/1
  v/1 -> Demux/1

== system Assignment_2_Spatial_Robotics/Nonlinear 6DoF ROV model (Quaternions)/Rigid-body Coriolis and centripetal matrix/Skew Symmetrical Operator ==
  v : Inport
  Constant : Constant  Value=0
  Create 3x3 Matrix : sharedutil/Create 3x3 Matrix  aMode=aMode
  Demux : Demux  Outputs=3
      settings: DisplayOption=none
  Gain : Gain  Gain=-1  SaturateOnIntegerOverflow=on  OutDataTypeStr=Inherit: Same as input  ParamDataTypeStr=Inherit: Same as input
  Gain1 : Gain  Gain=-1  SaturateOnIntegerOverflow=on  OutDataTypeStr=Inherit: Same as input  ParamDataTypeStr=Inherit: Same as input
  Gain2 : Gain  Gain=-1  SaturateOnIntegerOverflow=on  OutDataTypeStr=Inherit: Same as input  ParamDataTypeStr=Inherit: Same as input
  S(V) : Outport  VectorParamsAs1DForOutWhenUnconnected=off
  wires:
  Constant/1 -> Create 3x3 Matrix/1, Create 3x3 Matrix/9, Create 3x3 Matrix/5
  Demux/1 -> Gain/1, Create 3x3 Matrix/8  "v(1)"
  Demux/2 -> Gain1/1, Create 3x3 Matrix/3  "v(2)"
  Demux/3 -> Gain2/1, Create 3x3 Matrix/4  "v(3)"
  Gain/1 -> Create 3x3 Matrix/6  "-v(1)"
  Gain1/1 -> Create 3x3 Matrix/7  "-v(2)"
  Gain2/1 -> Create 3x3 Matrix/2  "-v(3)"
  Create 3x3 Matrix/1 -> S(V)/1
  v/1 -> Demux/1

== system Assignment_2_Spatial_Robotics/Nonlinear 6DoF ROV model (Quaternions)/Rigid-body Coriolis and centripetal matrix/Skew Symmetrical Operator  ==
  v : Inport
  Constant : Constant  Value=0
  Create 3x3 Matrix : sharedutil/Create 3x3 Matrix  aMode=aMode
  Demux : Demux  Outputs=3
      settings: DisplayOption=none
  Gain : Gain  Gain=-1  SaturateOnIntegerOverflow=on  OutDataTypeStr=Inherit: Same as input  ParamDataTypeStr=Inherit: Same as input
  Gain1 : Gain  Gain=-1  SaturateOnIntegerOverflow=on  OutDataTypeStr=Inherit: Same as input  ParamDataTypeStr=Inherit: Same as input
  Gain2 : Gain  Gain=-1  SaturateOnIntegerOverflow=on  OutDataTypeStr=Inherit: Same as input  ParamDataTypeStr=Inherit: Same as input
  S(V) : Outport  VectorParamsAs1DForOutWhenUnconnected=off
  wires:
  v/1 -> Demux/1
  Create 3x3 Matrix/1 -> S(V)/1
  Gain2/1 -> Create 3x3 Matrix/2  "-v(3)"
  Gain1/1 -> Create 3x3 Matrix/7  "-v(2)"
  Gain/1 -> Create 3x3 Matrix/6  "-v(1)"
  Demux/3 -> Create 3x3 Matrix/4, Gain2/1  "v(3)"
  Demux/2 -> Create 3x3 Matrix/3, Gain1/1  "v(2)"
  Demux/1 -> Create 3x3 Matrix/8, Gain/1  "v(1)"
  Constant/1 -> Create 3x3 Matrix/5, Create 3x3 Matrix/9, Create 3x3 Matrix/1

== system Assignment_2_Spatial_Robotics/Nonlinear 6DoF ROV model (Quaternions)/Rigid-body Coriolis and centripetal matrix/Skew Symmetrical Operator   ==
  v : Inport
  Constant : Constant  Value=0
  Create 3x3 Matrix : sharedutil/Create 3x3 Matrix  aMode=aMode
  Demux : Demux  Outputs=3
      settings: DisplayOption=none
  Gain : Gain  Gain=-1  SaturateOnIntegerOverflow=on  OutDataTypeStr=Inherit: Same as input  ParamDataTypeStr=Inherit: Same as input
  Gain1 : Gain  Gain=-1  SaturateOnIntegerOverflow=on  OutDataTypeStr=Inherit: Same as input  ParamDataTypeStr=Inherit: Same as input
  Gain2 : Gain  Gain=-1  SaturateOnIntegerOverflow=on  OutDataTypeStr=Inherit: Same as input  ParamDataTypeStr=Inherit: Same as input
  S(V) : Outport  VectorParamsAs1DForOutWhenUnconnected=off
  wires:
  Constant/1 -> Create 3x3 Matrix/1, Create 3x3 Matrix/9, Create 3x3 Matrix/5
  Demux/1 -> Gain/1, Create 3x3 Matrix/8  "v(1)"
  Demux/2 -> Gain1/1, Create 3x3 Matrix/3  "v(2)"
  Demux/3 -> Gain2/1, Create 3x3 Matrix/4  "v(3)"
  Gain/1 -> Create 3x3 Matrix/6  "-v(1)"
  Gain1/1 -> Create 3x3 Matrix/7  "-v(2)"
  Gain2/1 -> Create 3x3 Matrix/2  "-v(3)"
  Create 3x3 Matrix/1 -> S(V)/1
  v/1 -> Demux/1

== system Assignment_2_Spatial_Robotics/Nonlinear 6DoF ROV model (Quaternions)/6 DOF transformation/E1(q)/Skew Symmetrical Operator ==
  v : Inport
  Constant : Constant  Value=0
  Create 3x3 Matrix : sharedutil/Create 3x3 Matrix  aMode=aMode
  Demux : Demux  Outputs=3
      settings: DisplayOption=none
  Gain : Gain  Gain=-1  SaturateOnIntegerOverflow=on  OutDataTypeStr=Inherit: Same as input  ParamDataTypeStr=Inherit: Same as input
  Gain1 : Gain  Gain=-1  SaturateOnIntegerOverflow=on  OutDataTypeStr=Inherit: Same as input  ParamDataTypeStr=Inherit: Same as input
  Gain2 : Gain  Gain=-1  SaturateOnIntegerOverflow=on  OutDataTypeStr=Inherit: Same as input  ParamDataTypeStr=Inherit: Same as input
  S(V) : Outport  VectorParamsAs1DForOutWhenUnconnected=off
  wires:
  Constant/1 -> Create 3x3 Matrix/1, Create 3x3 Matrix/9, Create 3x3 Matrix/5
  Demux/1 -> Gain/1, Create 3x3 Matrix/8  "v(1)"
  Demux/2 -> Gain1/1, Create 3x3 Matrix/3  "v(2)"
  Demux/3 -> Gain2/1, Create 3x3 Matrix/4  "v(3)"
  Gain/1 -> Create 3x3 Matrix/6  "-v(1)"
  Gain1/1 -> Create 3x3 Matrix/7  "-v(2)"
  Gain2/1 -> Create 3x3 Matrix/2  "-v(3)"
  Create 3x3 Matrix/1 -> S(V)/1
  v/1 -> Demux/1

== system Assignment_2_Spatial_Robotics/Nonlinear 6DoF ROV model (Quaternions)/6 DOF transformation/E2(q)/Skew Symmetrical Operator ==
  v : Inport
  Constant : Constant  Value=0
  Create 3x3 Matrix : sharedutil/Create 3x3 Matrix  aMode=aMode
  Demux : Demux  Outputs=3
      settings: DisplayOption=none
  Gain : Gain  Gain=-1  SaturateOnIntegerOverflow=on  OutDataTypeStr=Inherit: Same as input  ParamDataTypeStr=Inherit: Same as input
  Gain1 : Gain  Gain=-1  SaturateOnIntegerOverflow=on  OutDataTypeStr=Inherit: Same as input  ParamDataTypeStr=Inherit: Same as input
  Gain2 : Gain  Gain=-1  SaturateOnIntegerOverflow=on  OutDataTypeStr=Inherit: Same as input  ParamDataTypeStr=Inherit: Same as input
  S(V) : Outport  VectorParamsAs1DForOutWhenUnconnected=off
  wires:
  v/1 -> Demux/1
  Create 3x3 Matrix/1 -> S(V)/1
  Gain2/1 -> Create 3x3 Matrix/2  "-v(3)"
  Gain1/1 -> Create 3x3 Matrix/7  "-v(2)"
  Gain/1 -> Create 3x3 Matrix/6  "-v(1)"
  Demux/3 -> Create 3x3 Matrix/4, Gain2/1  "v(3)"
  Demux/2 -> Create 3x3 Matrix/3, Gain1/1  "v(2)"
  Demux/1 -> Create 3x3 Matrix/8, Gain/1  "v(1)"
  Constant/1 -> Create 3x3 Matrix/5, Create 3x3 Matrix/9, Create 3x3 Matrix/1

== matlab function Assignment_2_Spatial_Robotics/Nonlinear 6DoF ROV model (Quaternions)/NED -> LAT//LON/MATLAB Function ==
  data: ECEF input; LAT_LON output
function LAT_LON = ECEF_LAT_LON(ECEF)
    % Function to convert ECEF Coordinates to Lat/Lon Coordinate Frame
    %
    %   Input:  ECEF Coordinates (3x1) vector - x; y; z
    %
    %   Output: LAT/LON Coordinates (3x1) vector - lon; lat; h

    % Extract ECEF x,y,z
    x = ECEF(1,1);
    y = ECEF(2,1);
    z = ECEF(3,1);

    % Define WGS-84 Parameters
    a = 6378137.0;
    b = 6356752.3142;
    e = sqrt((a^2-b^2)/(a^2));
    e_prim = sqrt((a^2-b^2)/(b^2));
    f = (a-b)/a;
    e2 = 2*f - f^2;

    % Calculate Reused Variables
    a_sqr = a^2;
    b_sqr = b^2;

    % Calculate lat/lon
    p = sqrt(x^2 + y^2);
    theta = atan2((z*a),(p*b));
    lon = atan2(y,x);
    lat = atan2((z+(e_prim^2)*b*sin(theta)^3),(p-e2*a*cos(theta)^3));

    % Calculate N
    N = (a_sqr)/sqrt(a_sqr*cos(lat)^2 + b_sqr*sin(lat)^2);

    % Calculate h
    h = (p/cos(lat)) - N;

    LAT_LON = [lon; lat; h];

== matlab function Assignment_2_Spatial_Robotics/Nonlinear 6DoF ROV model (Quaternions)/NED -> LAT//LON/LAT//LON -> ECEF ==
  data: LAT_LON input; ECEF output
function ECEF = LAT_LON_ECEF(LAT_LON)
    % Function to convert LAT/LON Coordinates to ECEF Coordinate Frame
    % uses WGS-84 World Parameters
    %
    %   Input: Lat/Lon (3x1) vector - Lon; Lat; h
    %
    %   Output: ECEF Coordinate Vector (3x1) x;y;z

    % Define Variables
    lon = LAT_LON(1,1)*(pi/180);
    lat = LAT_LON(2,1)*(pi/180);
    h = LAT_LON(3,1);

    % Define WGS-84 Parameters
    a = 6378137.0;
    b = 6356752.3142;

    % Calculate Reused Variables
    a_sqr = a^2;
    b_sqr = b^2;
    c_lat = cos(lat);
    s_lat = sin(lat);
    c_lon = cos(lon);
    s_lon = sin(lon);

    % Calculate N
    N = (a_sqr)/sqrt(a_sqr*c_lat^2 + b_sqr*s_lat^2);

    % Calculate ECEF
    ECEF = [(N+h)*c_lat*c_lon;
            (N+h)*c_lat*s_lon;
            (((b_sqr/a_sqr)*N)+h)*s_lat];

== matlab function Assignment_2_Spatial_Robotics/Nonlinear 6DoF ROV model (Quaternions)/NED -> LAT//LON/NED->ECEF ==
  data: LAT_LON input; ECEF output; NED input; Re_n output
function [ECEF, Re_n]= NED_ECEF(LAT_LON, NED)
    % Function to convert NED Coordinates to ECEF Coordinate Frame
    %
    %   Input:  Lat/Lon (3x1) vector - Lon; Lat; h
    %           NED Coordinates (3x1) vector - x; y; z
    %
    %   Output: ECEF Coordinate Vector (3x1) x;y;z
    %           Rotation Matrix Re_n (3x3)

    % Index Lat and Lon
    lon = LAT_LON(1,1)*(pi/180);
    lat = LAT_LON(2,1)*(pi/180);

    % Calculate cosine and sine
    c_lat = cos(lat);
    s_lat = sin(lat);
    c_lon = cos(lon);
    s_lon = sin(lon);

    % Create Matrix Re_n
    Re_n = [-c_lon*s_lat,   -s_lon, -c_lon*c_lat;
            -s_lon*s_lat,   c_lon,  -s_lon*c_lat;
            c_lat,          0,      -s_lat      ];

    % Calculate ECEF
    ECEF = Re_n * NED;
